simulink model "PID_Controller"  (R2025b)
settings: Solver=ode8  StartTime=0.0  StopTime=10  FixedStep=0.01  RelTol=1e-6
InitFcn:
  | A = [0 1;-1 -0.2];
  | B = [0; 1];
  | C = [1 0];
  | D = 0;
settings Model: Creator=bala4krish  LastModifiedBy=MehrSystem
settings SolverCC: AlgebraicLoopSolver=TrustRegion
settings DebuggingCC: UnconnectedInputMsg=warning  UnconnectedOutputMsg=warning  UnconnectedLineMsg=warning
settings ModelReferenceCC: EnableRefExpFcnMdlSchedulingChecks=on
settings RTWCC: GPUComputeCapability=3.5

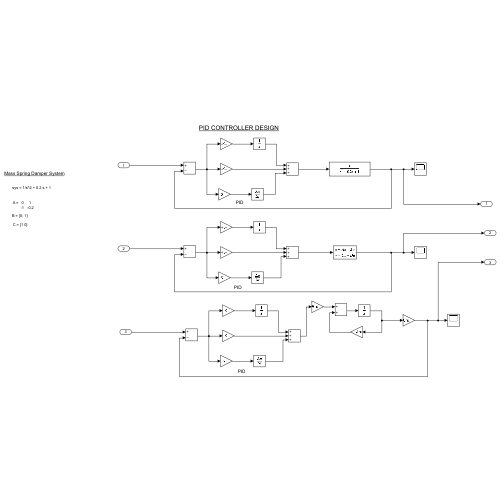
[thumbnail: Simulink's stored preview of the top-level diagram]
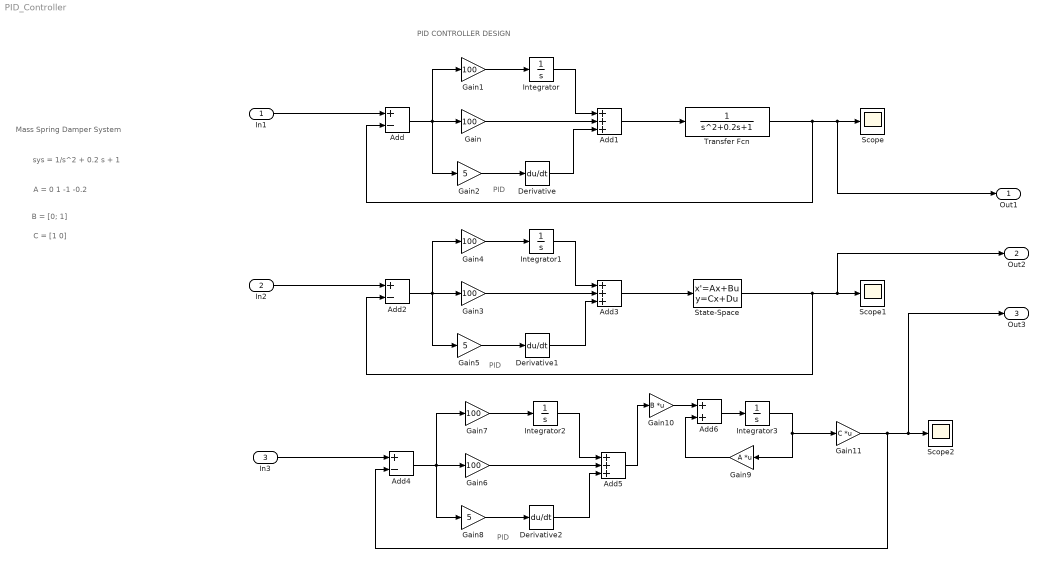
== system PID_Controller ==
  note: PID CONTROLLER DESIGN
  note: PID
  note: PID
  note: PID
  note: B = [0; 1]
  note: sys = 1/s^2 + 0.2 s + 1
  note: Mass Spring Damper System
  note: A =   0     1
      | 	-1   -0.2
  note: C = [1 0]
  In1 : Inport
  In2 : Inport  Port=2
  In3 : Inport  Port=3
  Add : Sum  Inputs=+-
  Add1 : Sum  Inputs=+++
  Add2 : Sum  Inputs=+-
  Add3 : Sum  Inputs=+++
  Add4 : Sum  Inputs=+-
  Add5 : Sum  Inputs=+++
  Add6 : Sum
  Derivative : Derivative
  Derivative1 : Derivative
  Derivative2 : Derivative
  Gain{,1,3..4,6..7} (6 alike) : Gain  Gain=100
  Gain10 : Gain  Gain=B  Multiplication=Matrix(K*u)
  Gain11 : Gain  Gain=C  Multiplication=Matrix(K*u)
  Gain2 : Gain  Gain=5
  Gain5 : Gain  Gain=5
  Gain8 : Gain  Gain=5
  Gain9 : Gain  Gain=A  Multiplication=Matrix(K*u)
  Integrator : Integrator  InitialCondition=1
  Integrator1 : Integrator  InitialCondition=1
  Integrator2 : Integrator  InitialCondition=1
  Integrator3 : Integrator
  Scope : Scope
      settings: ActiveDisplayYMinimum=-0.19506  ActiveDisplayYMaximum=1.75557
  Scope1 : Scope
      settings: ActiveDisplayYMinimum=-0.19516  ActiveDisplayYMaximum=1.75647
  Scope2 : Scope
      settings: ActiveDisplayYMinimum=-0.19516  ActiveDisplayYMaximum=1.75647  DataLoggingVariableName=ScopeData2
  State-Space : StateSpace  A=A  B=B  C=C  D=D  InitialCondition=0
  Transfer Fcn : TransferFcn  Denominator=[1 0.2 1]
  Out1 : Outport
  Out2 : Outport  Port=2
  Out3 : Outport  Port=3
  wires:
  Transfer Fcn/1 -> Add/2, Out1/1, Scope/1
  Add/1 -> Gain2/1, Gain1/1, Gain/1
  In1/1 -> Add/1
  Gain1/1 -> Integrator/1
  Integrator/1 -> Add1/1
  Gain/1 -> Add1/2
  Gain2/1 -> Derivative/1
  Derivative/1 -> Add1/3
  Add1/1 -> Transfer Fcn/1
  Add2/1 -> Gain5/1, Gain4/1, Gain3/1
  Integrator1/1 -> Add3/1
  Gain5/1 -> Derivative1/1
  Derivative1/1 -> Add3/3
  In2/1 -> Add2/1
  State-Space/1 -> Add2/2, Out2/1, Scope1/1
  Gain3/1 -> Add3/2
  Gain4/1 -> Integrator1/1
  Add3/1 -> State-Space/1
  Gain6/1 -> Add5/2
  Add4/1 -> Gain8/1, Gain7/1, Gain6/1
  Gain7/1 -> Integrator2/1
  Gain8/1 -> Derivative2/1
  Integrator2/1 -> Add5/1
  In3/1 -> Add4/1
  Derivative2/1 -> Add5/3
  Integrator3/1 -> Gain11/1, Gain9/1
  Gain10/1 -> Add6/1
  Add5/1 -> Gain10/1
  Gain9/1 -> Add6/2
  Add6/1 -> Integrator3/1
  Gain11/1 -> Add4/2, Out3/1, Scope2/1
